simulink model "step10_part1_ideal_neutral_model"  (R2024a)
settings: Solver=VariableStepAuto  StartTime=0.0  StopTime=10.0  RelTol=1e-3
libraries: fl_lib x40, ee_lib x14, nesl_utility x10
settings Model: Creator=Jonathan  LastModifiedBy=Jonathan
settings DebuggingCC: UnderspecifiedInitializationDetection=Classic  MergeDetectMultiDrivingBlocksExec=none
settings ModelReferenceCC: PropagateSignalLabelsOutOfModel=off

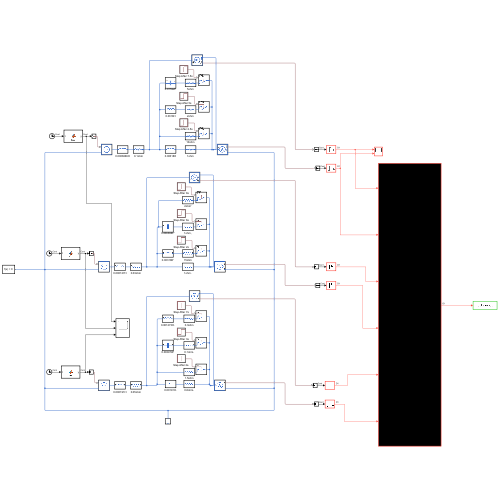
[thumbnail: Simulink's stored preview of the top-level diagram]
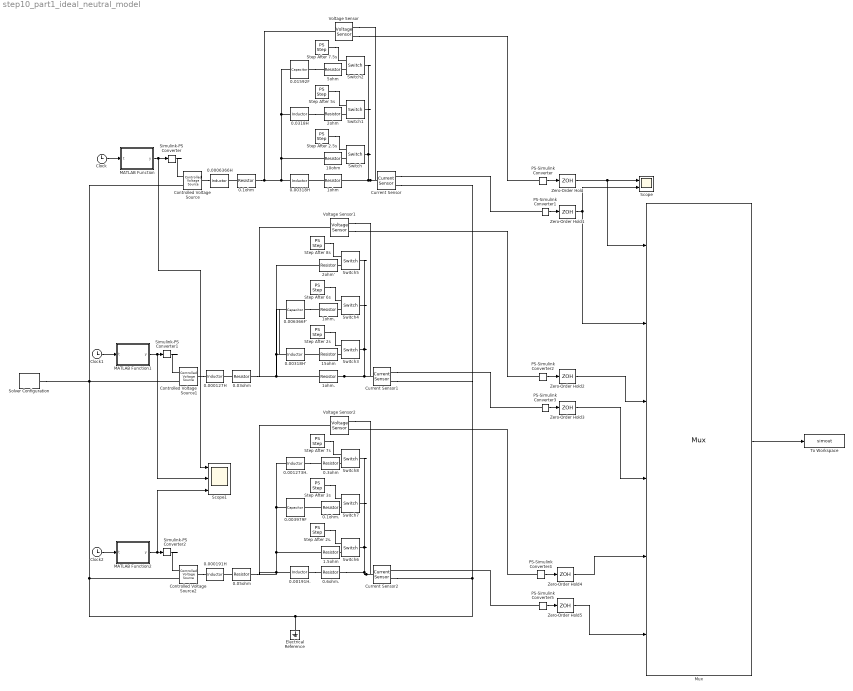
== system step10_part1_ideal_neutral_model ==
  0.000127H : ee_lib/Passive/Inductor  l=0.000127 H  enable_L_tol=ee.enum.toleranceApplication.none  L_tol=20  tol_distribution=ee.enum.toleranceDistribution.uniform  nSigma=4  r=0 Ohm  g=1e-9 1/Ohm  enable_operating_limits=ee.enum.enable.no  operating_limit_action=ee.enum.passive.reportOpLim.warn  max_working_current=1 A  power_rating=1 W  enable_faults=ee.enum.enable.no  fault_action=simscape.enum.assert.action.none  lambdaPercent=50  k_faulted=0.9999  turnsShort=ee.enum.passive.inductor.turnsShortOption.no  openCct=ee.enum.enable.no  groundShort=ee.enum.passive.inductor.groundShortOption.no  groundShortG=0 1/Ohm  tau_fault=1e-3 s  fault_trigger=ee.enum.faults.faultTrigger.temporal  t_fault=1 s  max_permissible_voltage=100 V  n_fail_on_voltage=1  max_permissible_current=1 A  t_fail_on_current=1 s  i_L_specify=off  i_L_priority=High  i_L=0 A  i_L_nominal_specify=off  i_L_nominal_value=1  i_L_nominal_unit=A  faulted_specify=off  faulted_priority=None  faulted=0
  0.000191H : ee_lib/Passive/Inductor  l=0.000191 H  enable_L_tol=ee.enum.toleranceApplication.none  L_tol=20  tol_distribution=ee.enum.toleranceDistribution.uniform  nSigma=4  r=0 Ohm  g=1e-9 1/Ohm  enable_operating_limits=ee.enum.enable.no  operating_limit_action=ee.enum.passive.reportOpLim.warn  max_working_current=1 A  power_rating=1 W  enable_faults=ee.enum.enable.no  fault_action=simscape.enum.assert.action.none  lambdaPercent=50  k_faulted=0.9999  turnsShort=ee.enum.passive.inductor.turnsShortOption.no  openCct=ee.enum.enable.no  groundShort=ee.enum.passive.inductor.groundShortOption.no  groundShortG=0 1/Ohm  tau_fault=1e-3 s  fault_trigger=ee.enum.faults.faultTrigger.temporal  t_fault=1 s  max_permissible_voltage=100 V  n_fail_on_voltage=1  max_permissible_current=1 A  t_fail_on_current=1 s  i_L_specify=off  i_L_priority=High  i_L=0 A  i_L_nominal_specify=off  i_L_nominal_value=1  i_L_nominal_unit=A  faulted_specify=off  faulted_priority=None  faulted=0
  0.0006366H : ee_lib/Passive/Inductor  l=0.0006366 H  enable_L_tol=ee.enum.toleranceApplication.none  L_tol=20  tol_distribution=ee.enum.toleranceDistribution.uniform  nSigma=4  r=0 Ohm  g=1e-9 1/Ohm  enable_operating_limits=ee.enum.enable.no  operating_limit_action=ee.enum.passive.reportOpLim.warn  max_working_current=1 A  power_rating=1 W  enable_faults=ee.enum.enable.no  fault_action=simscape.enum.assert.action.none  lambdaPercent=50  k_faulted=0.9999  turnsShort=ee.enum.passive.inductor.turnsShortOption.no  openCct=ee.enum.enable.no  groundShort=ee.enum.passive.inductor.groundShortOption.no  groundShortG=0 1/Ohm  tau_fault=1e-3 s  fault_trigger=ee.enum.faults.faultTrigger.temporal  t_fault=1 s  max_permissible_voltage=100 V  n_fail_on_voltage=1  max_permissible_current=1 A  t_fail_on_current=1 s  i_L_specify=off  i_L_priority=High  i_L=0 A  i_L_nominal_specify=off  i_L_nominal_value=1  i_L_nominal_unit=A  faulted_specify=off  faulted_priority=None  faulted=0
  0.001273H. : ee_lib/Passive/Inductor  l=0.001273 H  enable_L_tol=ee.enum.toleranceApplication.none  L_tol=20  tol_distribution=ee.enum.toleranceDistribution.uniform  nSigma=4  r=0 Ohm  g=1e-9 1/Ohm  enable_operating_limits=ee.enum.enable.no  operating_limit_action=ee.enum.passive.reportOpLim.warn  max_working_current=1 A  power_rating=1 W  enable_faults=ee.enum.enable.no  fault_action=simscape.enum.assert.action.none  lambdaPercent=50  k_faulted=0.9999  turnsShort=ee.enum.passive.inductor.turnsShortOption.no  openCct=ee.enum.enable.no  groundShort=ee.enum.passive.inductor.groundShortOption.no  groundShortG=0 1/Ohm  tau_fault=1e-3 s  fault_trigger=ee.enum.faults.faultTrigger.temporal  t_fault=1 s  max_permissible_voltage=100 V  n_fail_on_voltage=1  max_permissible_current=1 A  t_fail_on_current=1 s  i_L_specify=off  i_L_priority=High  i_L=0 A  i_L_nominal_specify=off  i_L_nominal_value=1  i_L_nominal_unit=A  faulted_specify=off  faulted_priority=None  faulted=0
  0.00191H. : ee_lib/Passive/Inductor  l=0.00191 H  enable_L_tol=ee.enum.toleranceApplication.none  L_tol=20  tol_distribution=ee.enum.toleranceDistribution.uniform  nSigma=4  r=0 Ohm  g=1e-9 1/Ohm  enable_operating_limits=ee.enum.enable.no  operating_limit_action=ee.enum.passive.reportOpLim.warn  max_working_current=1 A  power_rating=1 W  enable_faults=ee.enum.enable.no  fault_action=simscape.enum.assert.action.none  lambdaPercent=50  k_faulted=0.9999  turnsShort=ee.enum.passive.inductor.turnsShortOption.no  openCct=ee.enum.enable.no  groundShort=ee.enum.passive.inductor.groundShortOption.no  groundShortG=0 1/Ohm  tau_fault=1e-3 s  fault_trigger=ee.enum.faults.faultTrigger.temporal  t_fault=1 s  max_permissible_voltage=100 V  n_fail_on_voltage=1  max_permissible_current=1 A  t_fail_on_current=1 s  i_L_specify=off  i_L_priority=High  i_L=0 A  i_L_nominal_specify=off  i_L_nominal_value=1  i_L_nominal_unit=A  faulted_specify=off  faulted_priority=None  faulted=0
  0.00318H : ee_lib/Passive/Inductor  l=0.00318 H  enable_L_tol=ee.enum.toleranceApplication.none  L_tol=20  tol_distribution=ee.enum.toleranceDistribution.uniform  nSigma=4  r=0 Ohm  g=1e-9 1/Ohm  enable_operating_limits=ee.enum.enable.no  operating_limit_action=ee.enum.passive.reportOpLim.warn  max_working_current=1 A  power_rating=1 W  enable_faults=ee.enum.enable.no  fault_action=simscape.enum.assert.action.none  lambdaPercent=50  k_faulted=0.9999  turnsShort=ee.enum.passive.inductor.turnsShortOption.no  openCct=ee.enum.enable.no  groundShort=ee.enum.passive.inductor.groundShortOption.no  groundShortG=0 1/Ohm  tau_fault=1e-3 s  fault_trigger=ee.enum.faults.faultTrigger.temporal  t_fault=1 s  max_permissible_voltage=100 V  n_fail_on_voltage=1  max_permissible_current=1 A  t_fail_on_current=1 s  i_L_specify=off  i_L_priority=High  i_L=0 A  i_L_nominal_specify=off  i_L_nominal_value=1  i_L_nominal_unit=A  faulted_specify=off  faulted_priority=None  faulted=0
  0.00318H' : ee_lib/Passive/Inductor  l=0.00318 H  enable_L_tol=ee.enum.toleranceApplication.none  L_tol=20  tol_distribution=ee.enum.toleranceDistribution.uniform  nSigma=4  r=0 Ohm  g=1e-9 1/Ohm  enable_operating_limits=ee.enum.enable.no  operating_limit_action=ee.enum.passive.reportOpLim.warn  max_working_current=1 A  power_rating=1 W  enable_faults=ee.enum.enable.no  fault_action=simscape.enum.assert.action.none  lambdaPercent=50  k_faulted=0.9999  turnsShort=ee.enum.passive.inductor.turnsShortOption.no  openCct=ee.enum.enable.no  groundShort=ee.enum.passive.inductor.groundShortOption.no  groundShortG=0 1/Ohm  tau_fault=1e-3 s  fault_trigger=ee.enum.faults.faultTrigger.temporal  t_fault=1 s  max_permissible_voltage=100 V  n_fail_on_voltage=1  max_permissible_current=1 A  t_fail_on_current=1 s  i_L_specify=off  i_L_priority=High  i_L=0 A  i_L_nominal_specify=off  i_L_nominal_value=1  i_L_nominal_unit=A  faulted_specify=off  faulted_priority=None  faulted=0
  0.003979F : fl_lib/Electrical/Electrical Elements/Capacitor  c=0.003979 F  r=1e-6 Ohm  g=0 1/Ohm  i_specify=off  i_priority=None  i=0 A  i_nominal_specify=off  i_nominal_value=1  i_nominal_unit=A  v_specify=off  v_priority=None  v=0 V  v_nominal_specify=off  v_nominal_value=1  v_nominal_unit=V  vc_specify=off  vc_priority=High  vc=0 V  vc_nominal_specify=off  vc_nominal_value=1  vc_nominal_unit=V
  0.006366F' : fl_lib/Electrical/Electrical Elements/Capacitor  c=0.006366 F  r=1e-6 Ohm  g=0 1/Ohm  i_specify=off  i_priority=None  i=0 A  i_nominal_specify=off  i_nominal_value=1  i_nominal_unit=A  v_specify=off  v_priority=None  v=0 V  v_nominal_specify=off  v_nominal_value=1  v_nominal_unit=V  vc_specify=off  vc_priority=High  vc=0 V  vc_nominal_specify=off  vc_nominal_value=1  vc_nominal_unit=V
  0.01592F : fl_lib/Electrical/Electrical Elements/Capacitor  c=0.01592 F  r=1e-6 Ohm  g=0 1/Ohm  i_specify=off  i_priority=None  i=0 A  i_nominal_specify=off  i_nominal_value=1  i_nominal_unit=A  v_specify=off  v_priority=None  v=0 V  v_nominal_specify=off  v_nominal_value=1  v_nominal_unit=V  vc_specify=off  vc_priority=High  vc=0 V  vc_nominal_specify=off  vc_nominal_value=1  vc_nominal_unit=V
  0.0318H : ee_lib/Passive/Inductor  l=0.0318 H  enable_L_tol=ee.enum.toleranceApplication.none  L_tol=20  tol_distribution=ee.enum.toleranceDistribution.uniform  nSigma=4  r=0 Ohm  g=1e-9 1/Ohm  enable_operating_limits=ee.enum.enable.no  operating_limit_action=ee.enum.passive.reportOpLim.warn  max_working_current=1 A  power_rating=1 W  enable_faults=ee.enum.enable.no  fault_action=simscape.enum.assert.action.none  lambdaPercent=50  k_faulted=0.9999  turnsShort=ee.enum.passive.inductor.turnsShortOption.no  openCct=ee.enum.enable.no  groundShort=ee.enum.passive.inductor.groundShortOption.no  groundShortG=0 1/Ohm  tau_fault=1e-3 s  fault_trigger=ee.enum.faults.faultTrigger.temporal  t_fault=1 s  max_permissible_voltage=100 V  n_fail_on_voltage=1  max_permissible_current=1 A  t_fail_on_current=1 s  i_L_specify=off  i_L_priority=High  i_L=0 A  i_L_nominal_specify=off  i_L_nominal_value=1  i_L_nominal_unit=A  faulted_specify=off  faulted_priority=None  faulted=0
  0.03ohm : ee_lib/Passive/Resistor  R=0.03 Ohm  enable_R_tol=ee.enum.toleranceApplication.none  R_tol=5  tol_distribution=ee.enum.toleranceDistribution.uniform  nSigma=4  enable_operating_limits=ee.enum.enable.no  operating_limit_action=ee.enum.passive.reportOpLim.warn  power_rating=1 W  max_working_voltage=100 V  enable_faults=ee.enum.enable.no  fault_action=simscape.enum.assert.action.none  R_faulted=inf Ohm  fault_trigger=ee.enum.faults.faultTrigger.temporal  t_fault=1 s  max_permissible_current=1 A  t_fail_on_current=1 s  noise_mode=ee.enum.sources.noise.Disabled  Tdevice=25 degC  sample_time=1e-3 s  repeatability=ee.enum.ic.repeatability.notRepeatable  user_seed=0  auto_seed=545404223  faulted_specify=off  faulted_priority=None  faulted=0  power_derating_T1=70 degC  power_derating_T2=155 degC  operating_temperature_range_vec=[-50, 150] degC  alpha=3.93e-3 1/K  Tmeas=25 degC  thermal_mass=100 J/K  temperature_specify=off  temperature_priority=High  temperature=298.15 K  temperature_nominal_specify=off  temperature_nominal_value=1  temperature_nominal_unit=K
  0.05ohm : ee_lib/Passive/Resistor  R=0.05 Ohm  enable_R_tol=ee.enum.toleranceApplication.none  R_tol=5  tol_distribution=ee.enum.toleranceDistribution.uniform  nSigma=4  enable_operating_limits=ee.enum.enable.no  operating_limit_action=ee.enum.passive.reportOpLim.warn  power_rating=1 W  max_working_voltage=100 V  enable_faults=ee.enum.enable.no  fault_action=simscape.enum.assert.action.none  R_faulted=inf Ohm  fault_trigger=ee.enum.faults.faultTrigger.temporal  t_fault=1 s  max_permissible_current=1 A  t_fail_on_current=1 s  noise_mode=ee.enum.sources.noise.Disabled  Tdevice=25 degC  sample_time=1e-3 s  repeatability=ee.enum.ic.repeatability.notRepeatable  user_seed=0  auto_seed=2715962282  faulted_specify=off  faulted_priority=None  faulted=0  power_derating_T1=70 degC  power_derating_T2=155 degC  operating_temperature_range_vec=[-50, 150] degC  alpha=3.93e-3 1/K  Tmeas=25 degC  thermal_mass=100 J/K  temperature_specify=off  temperature_priority=High  temperature=298.15 K  temperature_nominal_specify=off  temperature_nominal_value=1  temperature_nominal_unit=K
  0.1ohm : ee_lib/Passive/Resistor  R=0.1 Ohm  enable_R_tol=ee.enum.toleranceApplication.none  R_tol=5  tol_distribution=ee.enum.toleranceDistribution.uniform  nSigma=4  enable_operating_limits=ee.enum.enable.no  operating_limit_action=ee.enum.passive.reportOpLim.warn  power_rating=1 W  max_working_voltage=100 V  enable_faults=ee.enum.enable.no  fault_action=simscape.enum.assert.action.none  R_faulted=inf Ohm  fault_trigger=ee.enum.faults.faultTrigger.temporal  t_fault=1 s  max_permissible_current=1 A  t_fail_on_current=1 s  noise_mode=ee.enum.sources.noise.Disabled  Tdevice=25 degC  sample_time=1e-3 s  repeatability=ee.enum.ic.repeatability.notRepeatable  user_seed=0  auto_seed=3499211588  faulted_specify=off  faulted_priority=None  faulted=0  power_derating_T1=70 degC  power_derating_T2=155 degC  operating_temperature_range_vec=[-50, 150] degC  alpha=3.93e-3 1/K  Tmeas=25 degC  thermal_mass=100 J/K  temperature_specify=off  temperature_priority=High  temperature=298.15 K  temperature_nominal_specify=off  temperature_nominal_value=1  temperature_nominal_unit=K
  0.1ohm. : fl_lib/Electrical/Electrical Elements/Resistor  R=0.1 Ohm  i_specify=off  i_priority=None  i=0 A  i_nominal_specify=off  i_nominal_value=1  i_nominal_unit=A  v_specify=off  v_priority=None  v=0 V  v_nominal_specify=off  v_nominal_value=1  v_nominal_unit=V
  0.3ohm : fl_lib/Electrical/Electrical Elements/Resistor  R=0.3 Ohm  i_specify=off  i_priority=None  i=0 A  i_nominal_specify=off  i_nominal_value=1  i_nominal_unit=A  v_specify=off  v_priority=None  v=0 V  v_nominal_specify=off  v_nominal_value=1  v_nominal_unit=V
  0.6ohm. : fl_lib/Electrical/Electrical Elements/Resistor  R=0.6 Ohm  i_specify=off  i_priority=None  i=0 A  i_nominal_specify=off  i_nominal_value=1  i_nominal_unit=A  v_specify=off  v_priority=None  v=0 V  v_nominal_specify=off  v_nominal_value=1  v_nominal_unit=V
  1.5ohm : ee_lib/Passive/Resistor  R=1.5 Ohm  enable_R_tol=ee.enum.toleranceApplication.none  R_tol=5  tol_distribution=ee.enum.toleranceDistribution.uniform  nSigma=4  enable_operating_limits=ee.enum.enable.no  operating_limit_action=ee.enum.passive.reportOpLim.warn  power_rating=1 W  max_working_voltage=100 V  enable_faults=ee.enum.enable.no  fault_action=simscape.enum.assert.action.none  R_faulted=inf Ohm  fault_trigger=ee.enum.faults.faultTrigger.temporal  t_fault=1 s  max_permissible_current=1 A  t_fail_on_current=1 s  noise_mode=ee.enum.sources.noise.Disabled  Tdevice=25 degC  sample_time=1e-3 s  repeatability=ee.enum.ic.repeatability.notRepeatable  user_seed=0  auto_seed=418932850  faulted_specify=off  faulted_priority=None  faulted=0  power_derating_T1=70 degC  power_derating_T2=155 degC  operating_temperature_range_vec=[-50, 150] degC  alpha=3.93e-3 1/K  Tmeas=25 degC  thermal_mass=100 J/K  temperature_specify=off  temperature_priority=High  temperature=298.15 K  temperature_nominal_specify=off  temperature_nominal_value=1  temperature_nominal_unit=K
  10ohm : fl_lib/Electrical/Electrical Elements/Resistor  R=10 Ohm  i_specify=off  i_priority=None  i=0 A  i_nominal_specify=off  i_nominal_value=1  i_nominal_unit=A  v_specify=off  v_priority=None  v=0 V  v_nominal_specify=off  v_nominal_value=1  v_nominal_unit=V
  15ohm : fl_lib/Electrical/Electrical Elements/Resistor  R=0.2 Ohm  i_specify=off  i_priority=None  i=0 A  i_nominal_specify=off  i_nominal_value=1  i_nominal_unit=A  v_specify=off  v_priority=None  v=0 V  v_nominal_specify=off  v_nominal_value=1  v_nominal_unit=V
  1ohm : ee_lib/Passive/Resistor  R=1 Ohm  enable_R_tol=ee.enum.toleranceApplication.none  R_tol=5  tol_distribution=ee.enum.toleranceDistribution.uniform  nSigma=4  enable_operating_limits=ee.enum.enable.no  operating_limit_action=ee.enum.passive.reportOpLim.warn  power_rating=1 W  max_working_voltage=100 V  enable_faults=ee.enum.enable.no  fault_action=simscape.enum.assert.action.none  R_faulted=inf Ohm  fault_trigger=ee.enum.faults.faultTrigger.temporal  t_fault=1 s  max_permissible_current=1 A  t_fail_on_current=1 s  noise_mode=ee.enum.sources.noise.Disabled  Tdevice=25 degC  sample_time=1e-3 s  repeatability=ee.enum.ic.repeatability.notRepeatable  user_seed=0  auto_seed=3890346746  faulted_specify=off  faulted_priority=None  faulted=0  power_derating_T1=70 degC  power_derating_T2=155 degC  operating_temperature_range_vec=[-50, 150] degC  alpha=3.93e-3 1/K  Tmeas=25 degC  thermal_mass=100 J/K  temperature_specify=off  temperature_priority=High  temperature=298.15 K  temperature_nominal_specify=off  temperature_nominal_value=1  temperature_nominal_unit=K
  1ohm, : fl_lib/Electrical/Electrical Elements/Resistor  R=0.5 Ohm  i_specify=off  i_priority=None  i=0 A  i_nominal_specify=off  i_nominal_value=1  i_nominal_unit=A  v_specify=off  v_priority=None  v=0 V  v_nominal_specify=off  v_nominal_value=1  v_nominal_unit=V
  1ohm. : ee_lib/Passive/Resistor  R=0.8 Ohm  enable_R_tol=ee.enum.toleranceApplication.none  R_tol=5  tol_distribution=ee.enum.toleranceDistribution.uniform  nSigma=4  enable_operating_limits=ee.enum.enable.no  operating_limit_action=ee.enum.passive.reportOpLim.warn  power_rating=1 W  max_working_voltage=100 V  enable_faults=ee.enum.enable.no  fault_action=simscape.enum.assert.action.none  R_faulted=inf Ohm  fault_trigger=ee.enum.faults.faultTrigger.temporal  t_fault=1 s  max_permissible_current=1 A  t_fail_on_current=1 s  noise_mode=ee.enum.sources.noise.Disabled  Tdevice=25 degC  sample_time=1e-3 s  repeatability=ee.enum.ic.repeatability.notRepeatable  user_seed=0  auto_seed=3922919431  faulted_specify=off  faulted_priority=None  faulted=0  power_derating_T1=70 degC  power_derating_T2=155 degC  operating_temperature_range_vec=[-50, 150] degC  alpha=3.93e-3 1/K  Tmeas=25 degC  thermal_mass=100 J/K  temperature_specify=off  temperature_priority=High  temperature=298.15 K  temperature_nominal_specify=off  temperature_nominal_value=1  temperature_nominal_unit=K
  2ohm : fl_lib/Electrical/Electrical Elements/Resistor  R=2 Ohm  i_specify=off  i_priority=None  i=0 A  i_nominal_specify=off  i_nominal_value=1  i_nominal_unit=A  v_specify=off  v_priority=None  v=0 V  v_nominal_specify=off  v_nominal_value=1  v_nominal_unit=V
  2ohm' : fl_lib/Electrical/Electrical Elements/Resistor  R=2 Ohm  i_specify=off  i_priority=None  i=0 A  i_nominal_specify=off  i_nominal_value=1  i_nominal_unit=A  v_specify=off  v_priority=None  v=0 V  v_nominal_specify=off  v_nominal_value=1  v_nominal_unit=V
  5ohm : fl_lib/Electrical/Electrical Elements/Resistor  R=5 Ohm  i_specify=off  i_priority=None  i=0 A  i_nominal_specify=off  i_nominal_value=1  i_nominal_unit=A  v_specify=off  v_priority=None  v=0 V  v_nominal_specify=off  v_nominal_value=1  v_nominal_unit=V
  Clock : Clock
  Clock1 : Clock
  Clock2 : Clock
  Controlled Voltage Source : fl_lib/Electrical/Electrical Sources/Controlled Voltage Source
  Controlled Voltage Source1 : fl_lib/Electrical/Electrical Sources/Controlled Voltage Source
  Controlled Voltage Source2 : fl_lib/Electrical/Electrical Sources/Controlled Voltage Source
  Current Sensor : fl_lib/Electrical/Electrical Sensors/Current Sensor
  Current Sensor1 : fl_lib/Electrical/Electrical Sensors/Current Sensor
  Current Sensor2 : fl_lib/Electrical/Electrical Sensors/Current Sensor
  Electrical Reference : fl_lib/Electrical/Electrical Elements/Electrical Reference
  MATLAB Function : MATLAB Function  TreatAsAtomicUnit=on
  MATLAB Function1 : MATLAB Function  TreatAsAtomicUnit=on
  MATLAB Function2 : MATLAB Function  TreatAsAtomicUnit=on
  Mux : Mux  Inputs=6
  PS-Simulink Converter{,1..5} (6 alike) : nesl_utility/PS-Simulink Converter  PhysicalDomain=network_engine_domain  SubClassName=ps_output  LeftPortType=input  RightPortType=output  PseudoPeriodic=off  Frequencies=[]  VectorFormat=inherit  Unit=inherit  AffineConversion=off
  Scope : Scope  NumInputPorts=2
  Scope1 : Scope  NumInputPorts=3
  Simulink-PS Converter : nesl_utility/Simulink-PS Converter  PhysicalDomain=network_engine_domain  SubClassName=ps_input  LeftPortType=input  RightPortType=output  PseudoPeriodic=off  Frequencies=[]  NoiseDistribution=none  NoiseParameters=[]  Unit=1  AffineConversion=off  FilteringAndDerivatives=provide  SimscapeFilterOrder=1  InputFilterTimeConstant=0.001  UdotUserProvided=0
  Simulink-PS Converter1 : nesl_utility/Simulink-PS Converter  PhysicalDomain=network_engine_domain  SubClassName=ps_input  LeftPortType=input  RightPortType=output  PseudoPeriodic=off  Frequencies=[]  NoiseDistribution=none  NoiseParameters=[]  Unit=1  AffineConversion=off  FilteringAndDerivatives=provide  SimscapeFilterOrder=1  InputFilterTimeConstant=0.001  UdotUserProvided=0
  Simulink-PS Converter2 : nesl_utility/Simulink-PS Converter  PhysicalDomain=network_engine_domain  SubClassName=ps_input  LeftPortType=input  RightPortType=output  PseudoPeriodic=off  Frequencies=[]  NoiseDistribution=none  NoiseParameters=[]  Unit=1  AffineConversion=off  FilteringAndDerivatives=provide  SimscapeFilterOrder=1  InputFilterTimeConstant=0.001  UdotUserProvided=0
  Solver Configuration : nesl_utility/Solver Configuration  PhysicalDomain=network_engine_domain  SubClassName=solver  LeftPortType=input  RightPortType=generic  Tones=[]  Harmonics=[]  SimulateNoise=off  Profile=off  UseLocalSampling=off  EnableSwitchedLinearOptims=on  FrequencyDomain=off  UseCCode=off  RelTol=0.001  AbsTol=0.001  MinStep=1e-09  ToWorkspace=off  RevertToSquareIcSolve=off  NumHomotopyIterations=100  PhasorMode=off  PhasorModeNumHarmonics=1  ConsistencySolver=NEWTON_XTOL_AFTER_FTOL  IndexReductionMethod=DerivativeReplacement  DoDC=off  ResidualTolerance=1e-09  ConsistencyTolSource=GLOBAL  ConsistencyAbsTol=0.001  ConsistencyRelTol=0.001  ConsistencyTolFactor=0.001  UseLocalSolver=off  LocalSolverChoice=NE_BACKWARD_EULER_ADVANCER  ResolveIndetEquations=on  FunctionEvalNumThread=1  LocalSolverSampleTime=0.001  DoFixedCost=off  MaxNonlinIter=3  MaxModeIter=2  ComputeImpulses=off  ImpulseIterations=2  LinearAlgebra=auto  LinearAlgebraNumThread=0  EquationFormulation=NE_TIME_EF  DelaysMemoryBudget=1024  AutomaticFiltering=on  FilteringTimeConstant=0.001  PartitionStorageMethod=AS_NEEDED  PartitionMemoryBudget=1024  PartitionMethod=ROBUST  MultibodyUseLocalSolver=off  MultibodyLocalSolverChoice=ODE1  MultibodyLocalSolverSampleTime=0.001
  Step After 2.5s : fl_lib/Physical Signals/Sources/PS Step  step_time=2.5 s  initial_value=0  final_value=1
  Step After 2s : fl_lib/Physical Signals/Sources/PS Step  step_time=2 s  initial_value=0  final_value=1
  Step After 2s. : fl_lib/Physical Signals/Sources/PS Step  step_time=2 s  initial_value=0  final_value=1
  Step After 3s : fl_lib/Physical Signals/Sources/PS Step  step_time=3 s  initial_value=0  final_value=1
  Step After 5s : fl_lib/Physical Signals/Sources/PS Step  step_time=5 s  initial_value=0  final_value=1
  Step After 6s : fl_lib/Physical Signals/Sources/PS Step  step_time=6 s  initial_value=0  final_value=1
  Step After 7.5s : fl_lib/Physical Signals/Sources/PS Step  step_time=7.5 s  initial_value=0  final_value=1
  Step After 7s : fl_lib/Physical Signals/Sources/PS Step  step_time=7 s  initial_value=0  final_value=1
  Step After 8s : fl_lib/Physical Signals/Sources/PS Step  step_time=8 s  initial_value=0  final_value=1
  Switch{,1..8} (9 alike) : fl_lib/Electrical/Electrical Elements/Switch  R_closed=0.01 Ohm  G_open=1e-8 1/Ohm  Threshold=0.5  i_specify=off  i_priority=None  i=0 A  i_nominal_specify=off  i_nominal_value=1  i_nominal_unit=A  v_specify=off  v_priority=None  v=0 V  v_nominal_specify=off  v_nominal_value=1  v_nominal_unit=V
  To Workspace : ToWorkspace  VariableName=simout  SaveFormat=Timeseries  SampleTime=1/8192
      settings: MaxDataPoints=81920
  Voltage Sensor : fl_lib/Electrical/Electrical Sensors/Voltage Sensor
  Voltage Sensor1 : fl_lib/Electrical/Electrical Sensors/Voltage Sensor
  Voltage Sensor2 : fl_lib/Electrical/Electrical Sensors/Voltage Sensor
  Zero-Order Hold{,1..5} (6 alike) : ZeroOrderHold  SampleTime=1/10000
  wires:
  PS-Simulink Converter/1 -> Zero-Order Hold/1
  Zero-Order Hold/1 -> Scope/1, Mux/1
  Zero-Order Hold1/1 -> Mux/2, Scope/2
  PS-Simulink Converter1/1 -> Zero-Order Hold1/1
  Mux/1 -> To Workspace/1
  Clock/1 -> MATLAB Function/1(t)
  MATLAB Function/1(y) -> Scope1/1, Simulink-PS Converter/1
  MATLAB Function1/1(y) -> Scope1/2, Simulink-PS Converter1/1
  Clock1/1 -> MATLAB Function1/1(t)
  PS-Simulink Converter2/1 -> Zero-Order Hold2/1
  PS-Simulink Converter3/1 -> Zero-Order Hold3/1
  Zero-Order Hold2/1 -> Mux/3
  Zero-Order Hold3/1 -> Mux/4
  MATLAB Function2/1(y) -> Scope1/3, Simulink-PS Converter2/1
  Clock2/1 -> MATLAB Function2/1(t)
  PS-Simulink Converter5/1 -> Zero-Order Hold5/1
  PS-Simulink Converter4/1 -> Zero-Order Hold4/1
  Zero-Order Hold4/1 -> Mux/5
  Zero-Order Hold5/1 -> Mux/6
  connections:
  1ohm/LConn1 -- 0.00318H/RConn1
  Solver Configuration/RConn1 -- Current Sensor1/RConn2 -- Current Sensor/RConn2 -- Current Sensor2/RConn2 -- Electrical Reference/LConn1 -- Controlled Voltage Source2/RConn2 -- Controlled Voltage Source1/RConn2 -- Controlled Voltage Source/RConn2
  Voltage Sensor/RConn1 -- PS-Simulink Converter/LConn1
  0.1ohm/RConn1 -- Voltage Sensor/LConn1 -- 0.00318H/LConn1 -- 0.01592F/LConn1 -- 0.0318H/LConn1 -- 10ohm/LConn1
  Current Sensor/LConn1 -- Voltage Sensor/RConn2 -- Switch2/LConn1 -- Switch1/LConn1 -- Switch/LConn1 -- 1ohm/RConn1
  Current Sensor/RConn1 -- PS-Simulink Converter1/LConn1
  0.1ohm/LConn1 -- 0.0006366H/RConn1
  Controlled Voltage Source/LConn1 -- 0.0006366H/LConn1
  Switch/RConn2 -- 10ohm/RConn1
  Step After 2.5s/RConn1 -- Switch/RConn1
  Step After 5s/RConn1 -- Switch1/RConn1
  Switch1/RConn2 -- 2ohm/RConn1
  Step After 7.5s/RConn1 -- Switch2/RConn1
  Switch2/RConn2 -- 5ohm/RConn1
  0.01592F/RConn1 -- 5ohm/LConn1
  0.0318H/RConn1 -- 2ohm/LConn1
  Simulink-PS Converter/RConn1 -- Controlled Voltage Source/RConn1
  1ohm./RConn1 -- Switch5/LConn1 -- Switch4/LConn1 -- Switch3/LConn1 -- Current Sensor1/LConn1 -- Voltage Sensor1/RConn2
  Step After 8s/RConn1 -- Switch5/RConn1
  Voltage Sensor1/RConn1 -- PS-Simulink Converter2/LConn1
  0.006366F'/RConn1 -- 1ohm,/LConn1
  Step After 6s/RConn1 -- Switch4/RConn1
  Controlled Voltage Source1/LConn1 -- 0.000127H/LConn1
  Switch5/RConn2 -- 2ohm'/RConn1
  Simulink-PS Converter1/RConn1 -- Controlled Voltage Source1/RConn1
  1ohm./LConn1 -- Voltage Sensor1/LConn1 -- 0.03ohm/RConn1 -- 2ohm'/LConn1 -- 0.006366F'/LConn1 -- 0.00318H'/LConn1
  0.03ohm/LConn1 -- 0.000127H/RConn1
  Switch4/RConn2 -- 1ohm,/RConn1
  Step After 2s/RConn1 -- Switch3/RConn1
  Switch3/RConn2 -- 15ohm/RConn1
  Current Sensor1/RConn1 -- PS-Simulink Converter3/LConn1
  Voltage Sensor2/RConn2 -- 0.6ohm./RConn1 -- Switch6/LConn1 -- Switch8/LConn1 -- Switch7/LConn1 -- Current Sensor2/LConn1
  Simulink-PS Converter2/RConn1 -- Controlled Voltage Source2/RConn1
  PS-Simulink Converter5/LConn1 -- Current Sensor2/RConn1
  Switch8/RConn2 -- 0.3ohm/RConn1
  0.05ohm/LConn1 -- 0.000191H/RConn1
  Step After 2s./RConn1 -- Switch6/RConn1
  Voltage Sensor2/LConn1 -- 0.05ohm/RConn1 -- 0.00191H./LConn1 -- 0.001273H./LConn1 -- 0.003979F/LConn1 -- 1.5ohm/LConn1
  PS-Simulink Converter4/LConn1 -- Voltage Sensor2/RConn1
  Step After 3s/RConn1 -- Switch7/RConn1
  Controlled Voltage Source2/LConn1 -- 0.000191H/LConn1
  Step After 7s/RConn1 -- Switch8/RConn1
  0.001273H./RConn1 -- 0.3ohm/LConn1
  15ohm/LConn1 -- 0.00318H'/RConn1
  Switch7/RConn2 -- 0.1ohm./RConn1
  Switch6/RConn2 -- 1.5ohm/RConn1
  0.00191H./RConn1 -- 0.6ohm./LConn1
  0.1ohm./LConn1 -- 0.003979F/RConn1

== matlab function step10_part1_ideal_neutral_model/MATLAB Function ==
  data: t input; y output
function y = fcn(t)

%=============================================================================================
% Generates a 230V peak square wave ramping linearly from 48 Hz to 52 Hz over 10s

    % Signal parameters
    %V_peak = 230 * sqrt(2); % Peak voltage magnitude (~325.27 V)
    %f_start = 48;           % Starting frequency (Hz)
    %f_end   = 52;           % Ending frequency (Hz)
    %T_total = 10;           % Packet duration (seconds)

    % Calculate instantaneous phase angle phi(t) in radians
    % phi(t) = 2 * pi * integral(f(t) dt) from 0 to t
    %f_ramp_rate = (f_end - f_start) / T_total; % 0.4 Hz/s
    %phi = 2 * pi * (f_start * t + 0.5 * f_ramp_rate * (t^2));

    % Generate symmetric square wave output using sign()
    %y = V_peak * sign(sin(phi));
    
    % Handle exact zero-crossing edge case to avoid outputting 0 V
    %if y == 0
        %y = V_peak;
    %end
%=============================================================================================

%=============================================================================================
    %Standard 50Hz sin wave
    %y = 230 * sqrt(2)*sin(2*pi()*50*t);
%=============================================================================================

%=============================================================================================
    % MATLAB Function Block: Generates 230V RMS (325.27V peak) sine wave
    % with linear frequency modulation between 48 Hz and 52 Hz over 10 seconds.
    
    A = 230 * sqrt(2);

    if t <= 10
        % Instantaneous frequency f(t) = 48 + 0.4*t
        % Phase phi = 2 * pi * integral(f(t) dt) = 2 * pi * (48*t + 0.2*t^2)
        phi = 2 * pi * (48 * t + 0.2 * t^2);
    else
        % Fixed frequency at 52 Hz after 10 seconds with continuous phase
        phi = 2 * pi * (52 * t - 20);
    end
    
    y = A * sin(phi);
%=============================================================================================
end

== matlab function step10_part1_ideal_neutral_model/MATLAB Function2 ==
  data: t input; y output
function y = fcn(t)

%=============================================================================================
% Generates a 230V peak square wave ramping linearly from 48 Hz to 52 Hz over 10s

    % Signal parameters
    %V_peak = 230 * sqrt(2); % Peak voltage magnitude (~325.27 V)
    %f_start = 48;           % Starting frequency (Hz)
    %f_end   = 52;           % Ending frequency (Hz)
    %T_total = 10;           % Packet duration (seconds)

    % Calculate instantaneous phase angle phi(t) in radians
    % phi(t) = 2 * pi * integral(f(t) dt) from 0 to t
    %f_ramp_rate = (f_end - f_start) / T_total; % 0.4 Hz/s
    %phi = 2 * pi * (f_start * t + 0.5 * f_ramp_rate * (t^2));

    % Generate symmetric square wave output using sign()
    %y = V_peak * sign(sin(phi));
    
    % Handle exact zero-crossing edge case to avoid outputting 0 V
    %if y == 0
        %y = V_peak;
    %end
%=============================================================================================

%=============================================================================================
    %Standard 50Hz sin wave
    %y = 230 * sqrt(2)*sin(2*pi()*50*t);
%=============================================================================================

%=============================================================================================
    % MATLAB Function Block: Generates 230V RMS (325.27V peak) sine wave
    % with linear frequency modulation between 48 Hz and 52 Hz over 10 seconds.
    
    A = 230 * sqrt(2);
if t <= 10
    % Instantaneous phase with +120 degree (+2*pi/3 rad) shift
    phi = 2 * pi * (48 * t + 0.2 * t^2) + (2 * pi / 3);
else
    phi = 2 * pi * (52 * t - 20) + (2 * pi / 3);
end

y = A * sin(phi);
%=============================================================================================
end

== matlab function step10_part1_ideal_neutral_model/MATLAB Function1 ==
  data: t input; y output
function y = fcn(t)

%=============================================================================================
% Generates a 230V peak square wave ramping linearly from 48 Hz to 52 Hz over 10s

    % Signal parameters
    %V_peak = 230 * sqrt(2); % Peak voltage magnitude (~325.27 V)
    %f_start = 48;           % Starting frequency (Hz)
    %f_end   = 52;           % Ending frequency (Hz)
    %T_total = 10;           % Packet duration (seconds)

    % Calculate instantaneous phase angle phi(t) in radians
    % phi(t) = 2 * pi * integral(f(t) dt) from 0 to t
    %f_ramp_rate = (f_end - f_start) / T_total; % 0.4 Hz/s
    %phi = 2 * pi * (f_start * t + 0.5 * f_ramp_rate * (t^2));

    % Generate symmetric square wave output using sign()
    %y = V_peak * sign(sin(phi));
    
    % Handle exact zero-crossing edge case to avoid outputting 0 V
    %if y == 0
        %y = V_peak;
    %end
%=============================================================================================

%=============================================================================================
    %Standard 50Hz sin wave
    %y = 230 * sqrt(2)*sin(2*pi()*50*t);
%=============================================================================================

%=============================================================================================
    % MATLAB Function Block: Generates 230V RMS (325.27V peak) sine wave
    % with linear frequency modulation between 48 Hz and 52 Hz over 10 seconds.
    
    A = 230 * sqrt(2);
if t <= 10
    % Instantaneous phase with -120 degree (-2*pi/3 rad) shift
    phi = 2 * pi * (48 * t + 0.2 * t^2) - (2 * pi / 3);
else
    phi = 2 * pi * (52 * t - 20) - (2 * pi / 3);
end

y = A * sin(phi);
%=============================================================================================
end
